simulink model "Acrobot_SwingUp"  (R2025b)
settings: Solver=ode45  StartTime=0.0  StopTime=Tstop  MaxStep=1e-3  RelTol=1e-7  AbsTol=1e-9
values from neighbouring files (symbols this model uses):
  c_switch = 5    [make_simulink_figures.m]    (also in run_simulink_models.m)
  gains = [20 2 3]    [make_simulink_figures.m]    (also in run_simulink_models.m)
  K = lqr(A, B, eye(4), cases{r, 3})    [run_simulink_models.m]
  x0 = [deg2rad(3); 0; 0; 0]    [make_simulink_figures.m]    (also in run_simulink_models.m = [deg2rad(d0); 0; 0])
undefined symbols (not defined in the file or in its folder): S
settings Model: Creator=bhargav_vemparala  LastModifiedBy=bhargav_vemparala

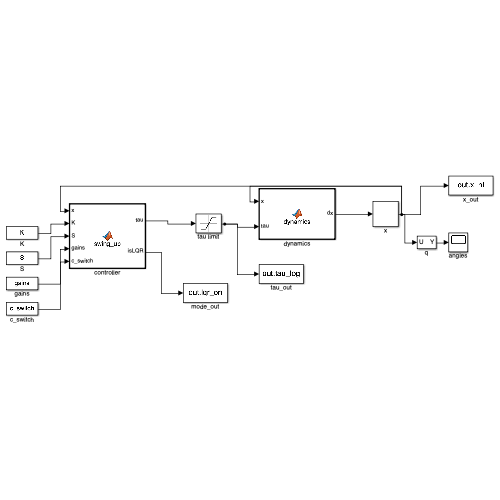
[thumbnail: Simulink's stored preview of the top-level diagram]
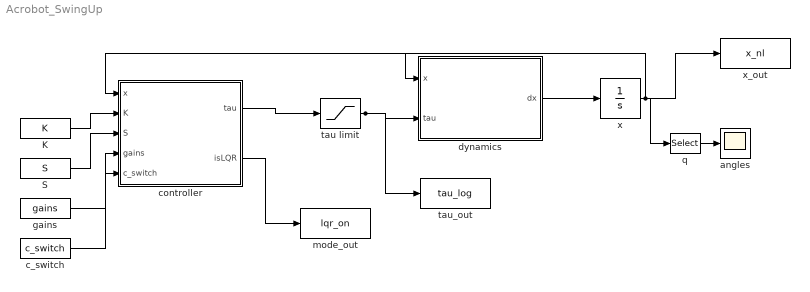
== system Acrobot_SwingUp ==
  K : Constant  Value=K
  S : Constant  Value=S
  angles : Scope
  c_switch : Constant  Value=c_switch
  controller : MATLAB Function  TreatAsAtomicUnit=on
  dynamics : MATLAB Function  TreatAsAtomicUnit=on
  gains : Constant  Value=gains
  mode_out : ToWorkspace  VariableName=lqr_on  SaveFormat=Timeseries  SampleTime=-1
  q : Selector  InputPortWidth=4  IndexOptions=Index vector (dialog)  Indices=[1 2]  OutputSizes=1
  tau limit : Saturate  UpperLimit=20  LowerLimit=-20
  tau_out : ToWorkspace  VariableName=tau_log  SaveFormat=Timeseries  SampleTime=-1
  x : Integrator  InitialCondition=x0
  x_out : ToWorkspace  VariableName=x_nl  SaveFormat=Timeseries  SampleTime=-1
  wires:
  dynamics/1(dx) -> x/1
  x/1 -> dynamics/1(x), x_out/1, q/1, controller/1(x)
  tau limit/1 -> dynamics/2(tau), tau_out/1
  q/1 -> angles/1
  K/1 -> controller/2(K)
  S/1 -> controller/3(S)
  gains/1 -> controller/4(gains)
  c_switch/1 -> controller/5(c_switch)
  controller/1(tau) -> tau limit/1
  controller/2(isLQR) -> mode_out/1

== matlab function Acrobot_SwingUp/controller ==
  data: x input; tau output; K input; S input; gains input; c_switch input; isLQR output
function [tau, isLQR] = swing_up(x, K, S, gains, c_switch)
%#codegen
% Hybrid controller: energy-pumping swing-up (partial feedback
% linearization) until x~'S x~ < c_switch, then the upright LQR.
q1 = x(1); q2 = x(2); d1 = x(3); d2 = x(4);
e = [mod(q1 - pi + pi, 2*pi) - pi; mod(q2 + pi, 2*pi) - pi; d1; d2];
isLQR = double((e'*S*e) < c_switch);
if isLQR > 0
    tau = -dot(K(:), e);
else
    c2 = cos(q2); s2 = sin(q2);
    m11 = 2.663 + 2*c2; m12 = 1.33 + c2; m22 = 1.33;
    E = 0.5*(m11*d1^2 + 2*m12*d1*d2 + m22*d2^2) - 14.715*cos(q1) - 9.81*cos(q1 + q2);
    h1 = -s2*(2*d1*d2 + d2^2) + 9.81*(1.5*sin(q1) + sin(q1 + q2));
    h2 = s2*d1^2 + 9.81*sin(q1 + q2);
    v = -gains(1)*(mod(q2 + pi, 2*pi) - pi) - gains(2)*d2 + gains(3)*d1*(E - 24.525);
    tau = (m22 - m12^2/m11)*v + h2 - m12*h1/m11;
end

== matlab function Acrobot_SwingUp/dynamics ==
  data: x input; dx output; tau input
function dx = dynamics(x, tau)
%#codegen
% Given acrobot model: M(q) qdd + C(q,qd) qd = tau_g(q) + B tau
q1 = x(1); q2 = x(2); d1 = x(3); d2 = x(4);
c2 = cos(q2); s2 = sin(q2);
M = [2.663 + 2*c2, 1.33 + c2; 1.33 + c2, 1.33];
Cqd = [-s2*(2*d1*d2 + d2^2); s2*d1^2];
tg = -9.81*[1.5*sin(q1) + sin(q1 + q2); sin(q1 + q2)];
qdd = M \ (tg + [0; tau] - Cqd);
dx = [d1; d2; qdd(1); qdd(2)];
